simulink model "ECG_Rhythm_PVC_Detection_v1_"  (R2019a)
settings: Solver=FixedStepDiscrete  StartTime=0.0  StopTime=10.0  FixedStep=1/360  RelTol=1e-3
libraries: dspfdesign x2, simulink x2, dspstat3 x1
settings Model: Creator=atif  LastModifiedBy=Admin

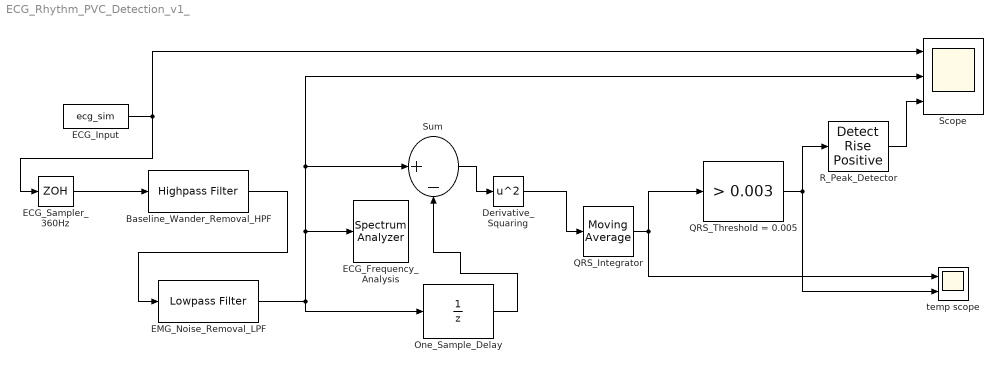
== system ECG_Rhythm_PVC_Detection_v1_ ==
  Baseline_Wander_Removal_HPF : dspfdesign/Highpass Filter  FilterType=FIR  DesignForMinimumOrder=on  FilterOrder=50  StopbandFrequency=0.1  PassbandFrequency=0.5  StopbandAttenuation=80  PassbandRipple=0.1  InheritSampleRate=off  SampleRate=360  SimulateUsing=Interpreted execution  roundingMode=Floor  coeffsDataTypeStr=fixdt(1,16)
      settings: SourceProductName=DSP System Toolbox
  Derivative_Squaring : Math  Operator=square  SaturateOnIntegerOverflow=on
  ECG_Frequency_Analysis : SpectrumAnalyzer
  ECG_Input : FromWorkspace  VariableName=ecg_sim  SampleTime=0  Interpolate=off  OutputAfterFinalValue=Holding final value
  ECG_Sampler_360Hz : ZeroOrderHold  SampleTime=1/360
  EMG_Noise_Removal_LPF : dspfdesign/Lowpass Filter  FilterType=FIR  DesignForMinimumOrder=on  FilterOrder=50  PassbandFrequency=40  StopbandFrequency=45  PassbandRipple=0.1  StopbandAttenuation=80  InheritSampleRate=off  SampleRate=360  SimulateUsing=Interpreted execution  roundingMode=Floor  coeffsDataTypeStr=fixdt(1,16)
  One_Sample_Delay : UnitDelay  SampleTime=1/360  HasFrameUpgradeWarning=on
  QRS_Integrator : dspstat3/Moving Average  Method=Sliding window  ForgettingFactorPort=off  SpecifyWindowLength=on  WindowLength=54  ForgettingFactor=0.9  SimulateUsing=Code generation
  QRS_Threshold = 0.005 : simulink/Logic and Bit Operations/Compare To Constant  relop=>  const=0.003  OutDataTypeStr=boolean
  R_Peak_Detector : simulink/Logic and Bit Operations/Detect Rise Positive  vinit=0  OutDataTypeStr=boolean
  Scope : Scope  NumInputPorts=3
  Sum : Sum  Inputs=|+-
  "temp scope " : Scope  NumInputPorts=2
  wires:
  ECG_Input/1 -> ECG_Sampler_360Hz/1, Scope/1
  Baseline_Wander_Removal_HPF/1 -> EMG_Noise_Removal_LPF/1
  ECG_Sampler_360Hz/1 -> Baseline_Wander_Removal_HPF/1
  One_Sample_Delay/1 -> Sum/2
  EMG_Noise_Removal_LPF/1 -> Scope/2, Sum/1, ECG_Frequency_Analysis/1, One_Sample_Delay/1
  Sum/1 -> Derivative_Squaring/1
  QRS_Integrator/1 -> "temp scope "/1, QRS_Threshold = 0.005/1
  Derivative_Squaring/1 -> QRS_Integrator/1
  QRS_Threshold = 0.005/1 -> R_Peak_Detector/1, "temp scope "/2
  R_Peak_Detector/1 -> Scope/3
